simulink model "dt_universalUR16e_dh"  (R2026a)
settings: Solver=daessc  StopTime=2.50
undefined symbols (not defined in the file or in its folder): X, Y, Z
libraries: nesl_utility x29, sm_lib x25
settings Model: Creator=User  LastModifiedBy=User

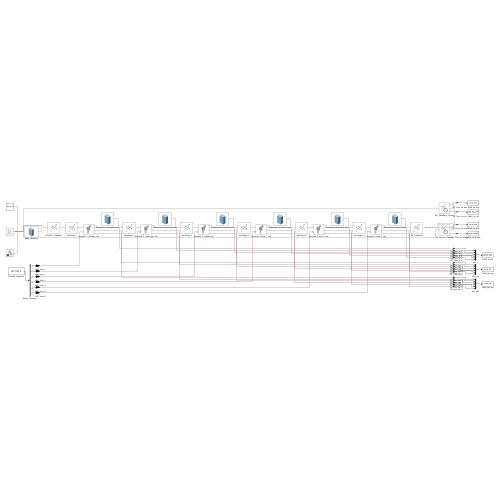
[thumbnail: Simulink's stored preview of the top-level diagram]
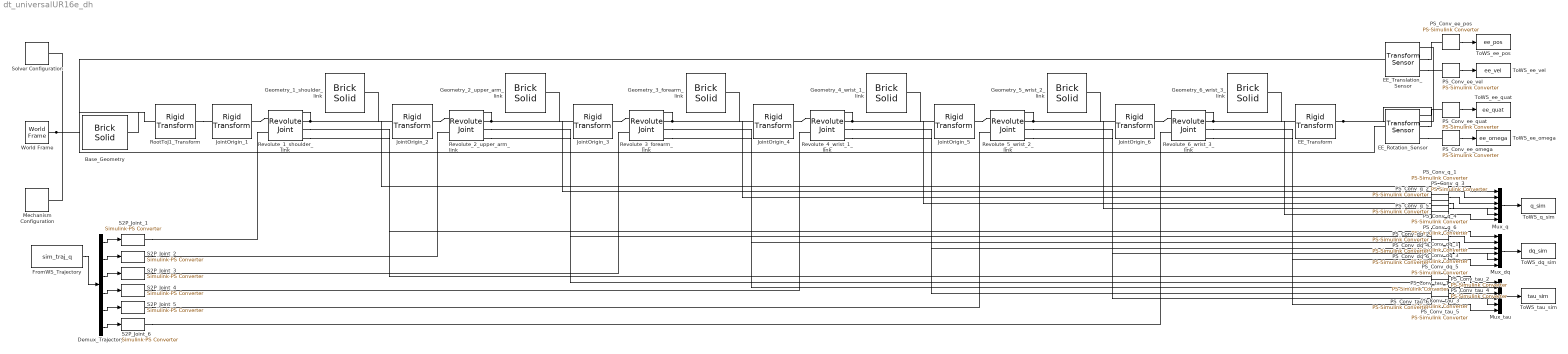
== system dt_universalUR16e_dh ==
  Base_Geometry : sm_lib/Body Elements/Brick Solid  BrickDimensions=[0.1, 0.1, 0.1]  BrickDimensionsUnits=m  ExportEntireGeometry=off  InertiaType=Custom  BasedOnType=Density  Density=1000  DensityUnits=kg/m^3  Mass=4.00000000  MassUnits=kg  CenterOfMass=[0.00000000, 0.00000000, 0.00000000]  CenterOfMassUnits=m  MomentsOfInertia=[0.00443000, 0.00443000, 0.00720000]  MomentsOfInertiaUnits=kg*m^2  ProductsOfInertia=[0, 0, 0]  ProductsOfInertiaUnits=kg*m^2  GraphicType=FromGeometry  MarkerShape=Sphere  MarkerSize=10  GraphicVisPropType=SimpleVisualProperties  GraphicDiffuseColor=[0.5 0.5 0.5]  GraphicOpacity=1  GraphicSpecularColor=[0.5 0.5 0.5 1.0]  GraphicAmbientColor=[0.15 0.15 0.15 1.0]  GraphicEmissiveColor=[0.0 0.0 0.0 1.0]  GraphicShininess=75  DoExposeReferenceFrame=on  SerializedFrames=<Frames/>
  Demux_Trajectory : Demux  Outputs=6
  EE_Rotation_Sensor : sm_lib/Frames and Transforms/Transform Sensor  MeasurementFrame=World  RotationSequence=XYX  SenseAngle=off  SenseAxis=off  SenseQ=on  SenseR=off  SenseRotationSequence=off  SenseOmegaX=off  SenseOmegaY=off  SenseOmegaZ=off  SenseOmega=on  SenseQDot=off  SenseRDot=off  SenseRotationSequenceDot=off  SenseAlphaX=off  SenseAlphaY=off  SenseAlphaZ=off  SenseAlpha=off  SenseQDDot=off  SenseRDDot=off  SenseX=off  SenseY=off  SenseZ=off  SenseXYZ=off  SenseRad=off  SenseAzim=off  SenseDist=off  SenseInc=off  SenseXDot=off  SenseYDot=off  SenseZDot=off  SenseXYZDot=off  SenseRadDot=off  SenseAzimDot=off  SenseDistDot=off  SenseIncDot=off  SenseXDDot=off  SenseYDDot=off  SenseZDDot=off  SenseXYZDDot=off  SenseRadDDot=off  SenseAzimDDot=off  SenseDistDDot=off  SenseIncDDot=off
  EE_Transform : sm_lib/Frames and Transforms/Rigid Transform  RotationMethod=ArbitraryAxis  FollAlignAxisA=+X  BaseAlignAxisA=+Y  FollAlignAxisB=+Y  BaseAlignAxisB=+Z  RotationStandardAxis=+Z  RotationAngle=3.1415926536  RotationAngleUnits=rad  RotationArbitraryAxis=[-0.0000000000, 1.0000000000, 0.0000000002]  RotationSequenceAxes=FollowerAxes  RotationSequence=XYX  RotationSequenceAngles=[0 0 0]  RotationSequenceAnglesUnits=deg  RotationMatrix=[1 0 0;0 1 0;0 0 1]  Quaternion=[1 0 0 0]  TranslationMethod=Cartesian  TranslationCartesianOffset=[-0.0000000000, -0.0000000000, -0.1165500000]  TranslationCartesianOffsetUnits=m  TranslationStandardAxis=+Z  TranslationStandardOffset=0  TranslationStandardOffsetUnits=m  TranslationROffset=0  TranslationROffsetUnits=m  TranslationThetaOffset=0  TranslationThetaOffsetUnits=deg  TranslationZOffset=0  TranslationZOffsetUnits=m
  EE_Translation_Sensor : sm_lib/Frames and Transforms/Transform Sensor  MeasurementFrame=World  RotationSequence=XYX  SenseAngle=off  SenseAxis=off  SenseQ=off  SenseR=off  SenseRotationSequence=off  SenseOmegaX=off  SenseOmegaY=off  SenseOmegaZ=off  SenseOmega=off  SenseQDot=off  SenseRDot=off  SenseRotationSequenceDot=off  SenseAlphaX=off  SenseAlphaY=off  SenseAlphaZ=off  SenseAlpha=off  SenseQDDot=off  SenseRDDot=off  SenseX=off  SenseY=off  SenseZ=off  SenseXYZ=on  SenseRad=off  SenseAzim=off  SenseDist=off  SenseInc=off  SenseXDot=off  SenseYDot=off  SenseZDot=off  SenseXYZDot=on  SenseRadDot=off  SenseAzimDot=off  SenseDistDot=off  SenseIncDot=off  SenseXDDot=off  SenseYDDot=off  SenseZDDot=off  SenseXYZDDot=off  SenseRadDDot=off  SenseAzimDDot=off  SenseDistDDot=off  SenseIncDDot=off
  FromWS_Trajectory : FromWorkspace  VariableName=sim_traj_q
  Geometry_1_shoulder_link : sm_lib/Body Elements/Brick Solid  BrickDimensions=[0.1, 0.1, 0.1]  BrickDimensionsUnits=m  ExportEntireGeometry=off  InertiaType=Custom  BasedOnType=Density  Density=1000  DensityUnits=kg/m^3  Mass=7.36900000  MassUnits=kg  CenterOfMass=[0.00000000, 0.00000000, 0.00000000]  CenterOfMassUnits=m  MomentsOfInertia=[0.02981926, 0.02981926, 0.02072531]  MomentsOfInertiaUnits=kg*m^2  ProductsOfInertia=[0.00000000, 0.00000000, 0.00000000]  ProductsOfInertiaUnits=kg*m^2  GraphicType=FromGeometry  MarkerShape=Sphere  MarkerSize=10  GraphicVisPropType=SimpleVisualProperties  GraphicDiffuseColor=[0.5 0.5 0.5]  GraphicOpacity=1  GraphicSpecularColor=[0.5 0.5 0.5 1.0]  GraphicAmbientColor=[0.15 0.15 0.15 1.0]  GraphicEmissiveColor=[0.0 0.0 0.0 1.0]  GraphicShininess=75  DoExposeReferenceFrame=on  SerializedFrames=<Frames/>
  Geometry_2_upper_arm_link : sm_lib/Body Elements/Brick Solid  BrickDimensions=[0.1, 0.1, 0.1]  BrickDimensionsUnits=m  ExportEntireGeometry=off  InertiaType=Custom  BasedOnType=Density  Density=1000  DensityUnits=kg/m^3  Mass=10.45000000  MassUnits=kg  CenterOfMass=[-0.23920000, 0.00000000, 0.17500000]  CenterOfMassUnits=m  MomentsOfInertia=[0.02939063, 0.21399986, 0.21399986]  MomentsOfInertiaUnits=kg*m^2  ProductsOfInertia=[0.00000000, -0.00000000, 0.00000000]  ProductsOfInertiaUnits=kg*m^2  GraphicType=FromGeometry  MarkerShape=Sphere  MarkerSize=10  GraphicVisPropType=SimpleVisualProperties  GraphicDiffuseColor=[0.5 0.5 0.5]  GraphicOpacity=1  GraphicSpecularColor=[0.5 0.5 0.5 1.0]  GraphicAmbientColor=[0.15 0.15 0.15 1.0]  GraphicEmissiveColor=[0.0 0.0 0.0 1.0]  GraphicShininess=75  DoExposeReferenceFrame=on  SerializedFrames=<Frames/>
  Geometry_3_forearm_link : sm_lib/Body Elements/Brick Solid  BrickDimensions=[0.1, 0.1, 0.1]  BrickDimensionsUnits=m  ExportEntireGeometry=off  InertiaType=Custom  BasedOnType=Density  Density=1000  DensityUnits=kg/m^3  Mass=4.32100000  MassUnits=kg  CenterOfMass=[-0.18000000, 0.00000000, 0.04000000]  CenterOfMassUnits=m  MomentsOfInertia=[0.01215281, 0.05274319, 0.05274319]  MomentsOfInertiaUnits=kg*m^2  ProductsOfInertia=[0.00000000, -0.00000000, 0.00000000]  ProductsOfInertiaUnits=kg*m^2  GraphicType=FromGeometry  MarkerShape=Sphere  MarkerSize=10  GraphicVisPropType=SimpleVisualProperties  GraphicDiffuseColor=[0.5 0.5 0.5]  GraphicOpacity=1  GraphicSpecularColor=[0.5 0.5 0.5 1.0]  GraphicAmbientColor=[0.15 0.15 0.15 1.0]  GraphicEmissiveColor=[0.0 0.0 0.0 1.0]  GraphicShininess=75  DoExposeReferenceFrame=on  SerializedFrames=<Frames/>
  Geometry_4_wrist_1_link : sm_lib/Body Elements/Brick Solid  BrickDimensions=[0.1, 0.1, 0.1]  BrickDimensionsUnits=m  ExportEntireGeometry=off  InertiaType=Custom  BasedOnType=Density  Density=1000  DensityUnits=kg/m^3  Mass=2.18000000  MassUnits=kg  CenterOfMass=[0.00000000, 0.00000000, 0.00000000]  CenterOfMassUnits=m  MomentsOfInertia=[0.00568162, 0.00568162, 0.00613125]  MomentsOfInertiaUnits=kg*m^2  ProductsOfInertia=[0.00000000, 0.00000000, 0.00000000]  ProductsOfInertiaUnits=kg*m^2  GraphicType=FromGeometry  MarkerShape=Sphere  MarkerSize=10  GraphicVisPropType=SimpleVisualProperties  GraphicDiffuseColor=[0.5 0.5 0.5]  GraphicOpacity=1  GraphicSpecularColor=[0.5 0.5 0.5 1.0]  GraphicAmbientColor=[0.15 0.15 0.15 1.0]  GraphicEmissiveColor=[0.0 0.0 0.0 1.0]  GraphicShininess=75  DoExposeReferenceFrame=on  SerializedFrames=<Frames/>
  Geometry_5_wrist_2_link : sm_lib/Body Elements/Brick Solid  BrickDimensions=[0.1, 0.1, 0.1]  BrickDimensionsUnits=m  ExportEntireGeometry=off  InertiaType=Custom  BasedOnType=Density  Density=1000  DensityUnits=kg/m^3  Mass=2.03300000  MassUnits=kg  CenterOfMass=[0.00000000, 0.00000000, 0.00000000]  CenterOfMassUnits=m  MomentsOfInertia=[0.00529850, 0.00529850, 0.00571781]  MomentsOfInertiaUnits=kg*m^2  ProductsOfInertia=[0.00000000, 0.00000000, 0.00000000]  ProductsOfInertiaUnits=kg*m^2  GraphicType=FromGeometry  MarkerShape=Sphere  MarkerSize=10  GraphicVisPropType=SimpleVisualProperties  GraphicDiffuseColor=[0.5 0.5 0.5]  GraphicOpacity=1  GraphicSpecularColor=[0.5 0.5 0.5 1.0]  GraphicAmbientColor=[0.15 0.15 0.15 1.0]  GraphicEmissiveColor=[0.0 0.0 0.0 1.0]  GraphicShininess=75  DoExposeReferenceFrame=on  SerializedFrames=<Frames/>
  Geometry_6_wrist_3_link : sm_lib/Body Elements/Brick Solid  BrickDimensions=[0.1, 0.1, 0.1]  BrickDimensionsUnits=m  ExportEntireGeometry=off  InertiaType=Custom  BasedOnType=Density  Density=1000  DensityUnits=kg/m^3  Mass=0.90700000  MassUnits=kg  CenterOfMass=[0.00000000, 0.00000000, -0.02500000]  CenterOfMassUnits=m  MomentsOfInertia=[0.00064813, 0.00064813, 0.00091834]  MomentsOfInertiaUnits=kg*m^2  ProductsOfInertia=[0.00000000, 0.00000000, 0.00000000]  ProductsOfInertiaUnits=kg*m^2  GraphicType=FromGeometry  MarkerShape=Sphere  MarkerSize=10  GraphicVisPropType=SimpleVisualProperties  GraphicDiffuseColor=[0.5 0.5 0.5]  GraphicOpacity=1  GraphicSpecularColor=[0.5 0.5 0.5 1.0]  GraphicAmbientColor=[0.15 0.15 0.15 1.0]  GraphicEmissiveColor=[0.0 0.0 0.0 1.0]  GraphicShininess=75  DoExposeReferenceFrame=on  SerializedFrames=<Frames/>
  JointOrigin_1 : sm_lib/Frames and Transforms/Rigid Transform  RotationMethod=None  FollAlignAxisA=+X  BaseAlignAxisA=+Y  FollAlignAxisB=+Y  BaseAlignAxisB=+Z  RotationStandardAxis=+Z  RotationAngle=0  RotationAngleUnits=deg  RotationArbitraryAxis=[0 0 1]  RotationSequenceAxes=FollowerAxes  RotationSequence=XYX  RotationSequenceAngles=[0 0 0]  RotationSequenceAnglesUnits=deg  RotationMatrix=[1 0 0;0 1 0;0 0 1]  Quaternion=[1 0 0 0]  TranslationMethod=Cartesian  TranslationCartesianOffset=[0.0000000000, 0.0000000000, 0.1807000000]  TranslationCartesianOffsetUnits=m  TranslationStandardAxis=+Z  TranslationStandardOffset=0  TranslationStandardOffsetUnits=m  TranslationROffset=0  TranslationROffsetUnits=m  TranslationThetaOffset=0  TranslationThetaOffsetUnits=deg  TranslationZOffset=0  TranslationZOffsetUnits=m
  JointOrigin_2 : sm_lib/Frames and Transforms/Rigid Transform  RotationMethod=ArbitraryAxis  FollAlignAxisA=+X  BaseAlignAxisA=+Y  FollAlignAxisB=+Y  BaseAlignAxisB=+Z  RotationStandardAxis=+Z  RotationAngle=1.5707963270  RotationAngleUnits=rad  RotationArbitraryAxis=[1.0000000000, 0.0000000000, 0.0000000000]  RotationSequenceAxes=FollowerAxes  RotationSequence=XYX  RotationSequenceAngles=[0 0 0]  RotationSequenceAnglesUnits=deg  RotationMatrix=[1 0 0;0 1 0;0 0 1]  Quaternion=[1 0 0 0]  TranslationMethod=Cartesian  TranslationCartesianOffset=[0.0000000000, 0.0000000000, 0.0000000000]  TranslationCartesianOffsetUnits=m  TranslationStandardAxis=+Z  TranslationStandardOffset=0  TranslationStandardOffsetUnits=m  TranslationROffset=0  TranslationROffsetUnits=m  TranslationThetaOffset=0  TranslationThetaOffsetUnits=deg  TranslationZOffset=0  TranslationZOffsetUnits=m
  JointOrigin_3 : sm_lib/Frames and Transforms/Rigid Transform  RotationMethod=None  FollAlignAxisA=+X  BaseAlignAxisA=+Y  FollAlignAxisB=+Y  BaseAlignAxisB=+Z  RotationStandardAxis=+Z  RotationAngle=0  RotationAngleUnits=deg  RotationArbitraryAxis=[0 0 1]  RotationSequenceAxes=FollowerAxes  RotationSequence=XYX  RotationSequenceAngles=[0 0 0]  RotationSequenceAnglesUnits=deg  RotationMatrix=[1 0 0;0 1 0;0 0 1]  Quaternion=[1 0 0 0]  TranslationMethod=Cartesian  TranslationCartesianOffset=[-0.4784000000, 0.0000000000, 0.0000000000]  TranslationCartesianOffsetUnits=m  TranslationStandardAxis=+Z  TranslationStandardOffset=0  TranslationStandardOffsetUnits=m  TranslationROffset=0  TranslationROffsetUnits=m  TranslationThetaOffset=0  TranslationThetaOffsetUnits=deg  TranslationZOffset=0  TranslationZOffsetUnits=m
  JointOrigin_4 : sm_lib/Frames and Transforms/Rigid Transform  RotationMethod=None  FollAlignAxisA=+X  BaseAlignAxisA=+Y  FollAlignAxisB=+Y  BaseAlignAxisB=+Z  RotationStandardAxis=+Z  RotationAngle=0  RotationAngleUnits=deg  RotationArbitraryAxis=[0 0 1]  RotationSequenceAxes=FollowerAxes  RotationSequence=XYX  RotationSequenceAngles=[0 0 0]  RotationSequenceAnglesUnits=deg  RotationMatrix=[1 0 0;0 1 0;0 0 1]  Quaternion=[1 0 0 0]  TranslationMethod=Cartesian  TranslationCartesianOffset=[-0.3600000000, 0.0000000000, 0.1741500000]  TranslationCartesianOffsetUnits=m  TranslationStandardAxis=+Z  TranslationStandardOffset=0  TranslationStandardOffsetUnits=m  TranslationROffset=0  TranslationROffsetUnits=m  TranslationThetaOffset=0  TranslationThetaOffsetUnits=deg  TranslationZOffset=0  TranslationZOffsetUnits=m
  JointOrigin_5 : sm_lib/Frames and Transforms/Rigid Transform  RotationMethod=ArbitraryAxis  FollAlignAxisA=+X  BaseAlignAxisA=+Y  FollAlignAxisB=+Y  BaseAlignAxisB=+Z  RotationStandardAxis=+Z  RotationAngle=1.5707963270  RotationAngleUnits=rad  RotationArbitraryAxis=[1.0000000000, 0.0000000000, 0.0000000000]  RotationSequenceAxes=FollowerAxes  RotationSequence=XYX  RotationSequenceAngles=[0 0 0]  RotationSequenceAnglesUnits=deg  RotationMatrix=[1 0 0;0 1 0;0 0 1]  Quaternion=[1 0 0 0]  TranslationMethod=Cartesian  TranslationCartesianOffset=[0.0000000000, -0.1198500000, -0.0000000000]  TranslationCartesianOffsetUnits=m  TranslationStandardAxis=+Z  TranslationStandardOffset=0  TranslationStandardOffsetUnits=m  TranslationROffset=0  TranslationROffsetUnits=m  TranslationThetaOffset=0  TranslationThetaOffsetUnits=deg  TranslationZOffset=0  TranslationZOffsetUnits=m
  JointOrigin_6 : sm_lib/Frames and Transforms/Rigid Transform  RotationMethod=ArbitraryAxis  FollAlignAxisA=+X  BaseAlignAxisA=+Y  FollAlignAxisB=+Y  BaseAlignAxisB=+Z  RotationStandardAxis=+Z  RotationAngle=1.5707963270  RotationAngleUnits=rad  RotationArbitraryAxis=[-1.0000000000, -0.0000000000, -0.0000000000]  RotationSequenceAxes=FollowerAxes  RotationSequence=XYX  RotationSequenceAngles=[0 0 0]  RotationSequenceAnglesUnits=deg  RotationMatrix=[1 0 0;0 1 0;0 0 1]  Quaternion=[1 0 0 0]  TranslationMethod=Cartesian  TranslationCartesianOffset=[0.0000000000, 0.1165500000, -0.0000000000]  TranslationCartesianOffsetUnits=m  TranslationStandardAxis=+Z  TranslationStandardOffset=0  TranslationStandardOffsetUnits=m  TranslationROffset=0  TranslationROffsetUnits=m  TranslationThetaOffset=0  TranslationThetaOffsetUnits=deg  TranslationZOffset=0  TranslationZOffsetUnits=m
  Mechanism Configuration : sm_lib/Utilities/Mechanism Configuration  UniformGravity=Constant  GravityVector=[0.0000000000, 0.0000000000, -9.8100000000]  GravityVectorUnits=m/s^2  LinearizationDelta=0.001  JointModeTransitionNonlinearIterations=2
  Mux_dq : Mux  Inputs=6
  Mux_q : Mux  Inputs=6
  Mux_tau : Mux  Inputs=6
  PS_Conv_dq_{1..6} (6 alike) : nesl_utility/PS-Simulink Converter  PhysicalDomain=network_engine_domain  SubClassName=ps_output  LeftPortType=input  RightPortType=output  PseudoPeriodic=off  Frequencies=[]  VectorFormat=inherit  Unit=inherit  AffineConversion=off
  PS_Conv_ee_omega : nesl_utility/PS-Simulink Converter  PhysicalDomain=network_engine_domain  SubClassName=ps_output  LeftPortType=input  RightPortType=output  PseudoPeriodic=off  Frequencies=[]  VectorFormat=inherit  Unit=inherit  AffineConversion=off
  PS_Conv_ee_pos : nesl_utility/PS-Simulink Converter  PhysicalDomain=network_engine_domain  SubClassName=ps_output  LeftPortType=input  RightPortType=output  PseudoPeriodic=off  Frequencies=[]  VectorFormat=inherit  Unit=inherit  AffineConversion=off
  PS_Conv_ee_quat : nesl_utility/PS-Simulink Converter  PhysicalDomain=network_engine_domain  SubClassName=ps_output  LeftPortType=input  RightPortType=output  PseudoPeriodic=off  Frequencies=[]  VectorFormat=inherit  Unit=inherit  AffineConversion=off
  PS_Conv_ee_vel : nesl_utility/PS-Simulink Converter  PhysicalDomain=network_engine_domain  SubClassName=ps_output  LeftPortType=input  RightPortType=output  PseudoPeriodic=off  Frequencies=[]  VectorFormat=inherit  Unit=inherit  AffineConversion=off
  PS_Conv_q_{1..6} (6 alike) : nesl_utility/PS-Simulink Converter  PhysicalDomain=network_engine_domain  SubClassName=ps_output  LeftPortType=input  RightPortType=output  PseudoPeriodic=off  Frequencies=[]  VectorFormat=inherit  Unit=inherit  AffineConversion=off
  PS_Conv_tau_{1..6} (6 alike) : nesl_utility/PS-Simulink Converter  PhysicalDomain=network_engine_domain  SubClassName=ps_output  LeftPortType=input  RightPortType=output  PseudoPeriodic=off  Frequencies=[]  VectorFormat=inherit  Unit=inherit  AffineConversion=off
  Revolute_1_shoulder_link : sm_lib/Joints/Revolute Joint  JointMode=Normal  CompositeWrenchDir=FollowerOnBase  CompositeWrenchFrame=BaseFrame  SenseConstraintForce=off  SenseConstraintTorque=off  SenseTotalForce=off  SenseTotalTorque=off  PositionTargetSpecify=off  PositionTargetPriority=High  PositionTargetValue=0  PositionTargetValueUnits=deg  VelocityTargetSpecify=off  VelocityTargetPriority=High  VelocityTargetValue=0  VelocityTargetValueUnits=deg/s  EquilibriumPosition=0  EquilibriumPositionUnits=deg  SpringStiffness=0  SpringStiffnessUnits=N*m/deg  DampingCoefficient=0  DampingCoefficientUnits=N*m/(deg/s)  LowerLimitSpecify=off  LowerLimitBound=-90  LowerLimitBoundUnits=deg  LowerLimitStiffness=1e4  LowerLimitStiffnessUnits=N*m/deg  LowerLimitDamping=10  LowerLimitDampingUnits=N*m/(deg/s)  LowerLimitTransitionRegionWidth=0.1  LowerLimitTransitionRegionWidthUnits=deg  UpperLimitSpecify=off  UpperLimitBound=90  UpperLimitBoundUnits=deg  UpperLimitStiffness=1e4  UpperLimitStiffnessUnits=N*m/deg  UpperLimitDamping=10  UpperLimitDampingUnits=N*m/(deg/s)  UpperLimitTransitionRegionWidth=0.1  UpperLimitTransitionRegionWidthUnits=deg  TorqueActuationMode=ComputedTorque  MotionActuationMode=InputMotion  SensePosition=on  SenseVelocity=on  SenseAcceleration=off  SenseTorqueForce=on  SenseLowerLimitTorqueForce=off  SenseUpperLimitTorqueForce=off
  Revolute_2_upper_arm_link : sm_lib/Joints/Revolute Joint  JointMode=Normal  CompositeWrenchDir=FollowerOnBase  CompositeWrenchFrame=BaseFrame  SenseConstraintForce=off  SenseConstraintTorque=off  SenseTotalForce=off  SenseTotalTorque=off  PositionTargetSpecify=off  PositionTargetPriority=High  PositionTargetValue=0  PositionTargetValueUnits=deg  VelocityTargetSpecify=off  VelocityTargetPriority=High  VelocityTargetValue=0  VelocityTargetValueUnits=deg/s  EquilibriumPosition=0  EquilibriumPositionUnits=deg  SpringStiffness=0  SpringStiffnessUnits=N*m/deg  DampingCoefficient=0  DampingCoefficientUnits=N*m/(deg/s)  LowerLimitSpecify=off  LowerLimitBound=-90  LowerLimitBoundUnits=deg  LowerLimitStiffness=1e4  LowerLimitStiffnessUnits=N*m/deg  LowerLimitDamping=10  LowerLimitDampingUnits=N*m/(deg/s)  LowerLimitTransitionRegionWidth=0.1  LowerLimitTransitionRegionWidthUnits=deg  UpperLimitSpecify=off  UpperLimitBound=90  UpperLimitBoundUnits=deg  UpperLimitStiffness=1e4  UpperLimitStiffnessUnits=N*m/deg  UpperLimitDamping=10  UpperLimitDampingUnits=N*m/(deg/s)  UpperLimitTransitionRegionWidth=0.1  UpperLimitTransitionRegionWidthUnits=deg  TorqueActuationMode=ComputedTorque  MotionActuationMode=InputMotion  SensePosition=on  SenseVelocity=on  SenseAcceleration=off  SenseTorqueForce=on  SenseLowerLimitTorqueForce=off  SenseUpperLimitTorqueForce=off
  Revolute_3_forearm_link : sm_lib/Joints/Revolute Joint  JointMode=Normal  CompositeWrenchDir=FollowerOnBase  CompositeWrenchFrame=BaseFrame  SenseConstraintForce=off  SenseConstraintTorque=off  SenseTotalForce=off  SenseTotalTorque=off  PositionTargetSpecify=off  PositionTargetPriority=High  PositionTargetValue=0  PositionTargetValueUnits=deg  VelocityTargetSpecify=off  VelocityTargetPriority=High  VelocityTargetValue=0  VelocityTargetValueUnits=deg/s  EquilibriumPosition=0  EquilibriumPositionUnits=deg  SpringStiffness=0  SpringStiffnessUnits=N*m/deg  DampingCoefficient=0  DampingCoefficientUnits=N*m/(deg/s)  LowerLimitSpecify=off  LowerLimitBound=-90  LowerLimitBoundUnits=deg  LowerLimitStiffness=1e4  LowerLimitStiffnessUnits=N*m/deg  LowerLimitDamping=10  LowerLimitDampingUnits=N*m/(deg/s)  LowerLimitTransitionRegionWidth=0.1  LowerLimitTransitionRegionWidthUnits=deg  UpperLimitSpecify=off  UpperLimitBound=90  UpperLimitBoundUnits=deg  UpperLimitStiffness=1e4  UpperLimitStiffnessUnits=N*m/deg  UpperLimitDamping=10  UpperLimitDampingUnits=N*m/(deg/s)  UpperLimitTransitionRegionWidth=0.1  UpperLimitTransitionRegionWidthUnits=deg  TorqueActuationMode=ComputedTorque  MotionActuationMode=InputMotion  SensePosition=on  SenseVelocity=on  SenseAcceleration=off  SenseTorqueForce=on  SenseLowerLimitTorqueForce=off  SenseUpperLimitTorqueForce=off
  Revolute_4_wrist_1_link : sm_lib/Joints/Revolute Joint  JointMode=Normal  CompositeWrenchDir=FollowerOnBase  CompositeWrenchFrame=BaseFrame  SenseConstraintForce=off  SenseConstraintTorque=off  SenseTotalForce=off  SenseTotalTorque=off  PositionTargetSpecify=off  PositionTargetPriority=High  PositionTargetValue=0  PositionTargetValueUnits=deg  VelocityTargetSpecify=off  VelocityTargetPriority=High  VelocityTargetValue=0  VelocityTargetValueUnits=deg/s  EquilibriumPosition=0  EquilibriumPositionUnits=deg  SpringStiffness=0  SpringStiffnessUnits=N*m/deg  DampingCoefficient=0  DampingCoefficientUnits=N*m/(deg/s)  LowerLimitSpecify=off  LowerLimitBound=-90  LowerLimitBoundUnits=deg  LowerLimitStiffness=1e4  LowerLimitStiffnessUnits=N*m/deg  LowerLimitDamping=10  LowerLimitDampingUnits=N*m/(deg/s)  LowerLimitTransitionRegionWidth=0.1  LowerLimitTransitionRegionWidthUnits=deg  UpperLimitSpecify=off  UpperLimitBound=90  UpperLimitBoundUnits=deg  UpperLimitStiffness=1e4  UpperLimitStiffnessUnits=N*m/deg  UpperLimitDamping=10  UpperLimitDampingUnits=N*m/(deg/s)  UpperLimitTransitionRegionWidth=0.1  UpperLimitTransitionRegionWidthUnits=deg  TorqueActuationMode=ComputedTorque  MotionActuationMode=InputMotion  SensePosition=on  SenseVelocity=on  SenseAcceleration=off  SenseTorqueForce=on  SenseLowerLimitTorqueForce=off  SenseUpperLimitTorqueForce=off
  Revolute_5_wrist_2_link : sm_lib/Joints/Revolute Joint  JointMode=Normal  CompositeWrenchDir=FollowerOnBase  CompositeWrenchFrame=BaseFrame  SenseConstraintForce=off  SenseConstraintTorque=off  SenseTotalForce=off  SenseTotalTorque=off  PositionTargetSpecify=off  PositionTargetPriority=High  PositionTargetValue=0  PositionTargetValueUnits=deg  VelocityTargetSpecify=off  VelocityTargetPriority=High  VelocityTargetValue=0  VelocityTargetValueUnits=deg/s  EquilibriumPosition=0  EquilibriumPositionUnits=deg  SpringStiffness=0  SpringStiffnessUnits=N*m/deg  DampingCoefficient=0  DampingCoefficientUnits=N*m/(deg/s)  LowerLimitSpecify=off  LowerLimitBound=-90  LowerLimitBoundUnits=deg  LowerLimitStiffness=1e4  LowerLimitStiffnessUnits=N*m/deg  LowerLimitDamping=10  LowerLimitDampingUnits=N*m/(deg/s)  LowerLimitTransitionRegionWidth=0.1  LowerLimitTransitionRegionWidthUnits=deg  UpperLimitSpecify=off  UpperLimitBound=90  UpperLimitBoundUnits=deg  UpperLimitStiffness=1e4  UpperLimitStiffnessUnits=N*m/deg  UpperLimitDamping=10  UpperLimitDampingUnits=N*m/(deg/s)  UpperLimitTransitionRegionWidth=0.1  UpperLimitTransitionRegionWidthUnits=deg  TorqueActuationMode=ComputedTorque  MotionActuationMode=InputMotion  SensePosition=on  SenseVelocity=on  SenseAcceleration=off  SenseTorqueForce=on  SenseLowerLimitTorqueForce=off  SenseUpperLimitTorqueForce=off
  Revolute_6_wrist_3_link : sm_lib/Joints/Revolute Joint  JointMode=Normal  CompositeWrenchDir=FollowerOnBase  CompositeWrenchFrame=BaseFrame  SenseConstraintForce=off  SenseConstraintTorque=off  SenseTotalForce=off  SenseTotalTorque=off  PositionTargetSpecify=off  PositionTargetPriority=High  PositionTargetValue=0  PositionTargetValueUnits=deg  VelocityTargetSpecify=off  VelocityTargetPriority=High  VelocityTargetValue=0  VelocityTargetValueUnits=deg/s  EquilibriumPosition=0  EquilibriumPositionUnits=deg  SpringStiffness=0  SpringStiffnessUnits=N*m/deg  DampingCoefficient=0  DampingCoefficientUnits=N*m/(deg/s)  LowerLimitSpecify=off  LowerLimitBound=-90  LowerLimitBoundUnits=deg  LowerLimitStiffness=1e4  LowerLimitStiffnessUnits=N*m/deg  LowerLimitDamping=10  LowerLimitDampingUnits=N*m/(deg/s)  LowerLimitTransitionRegionWidth=0.1  LowerLimitTransitionRegionWidthUnits=deg  UpperLimitSpecify=off  UpperLimitBound=90  UpperLimitBoundUnits=deg  UpperLimitStiffness=1e4  UpperLimitStiffnessUnits=N*m/deg  UpperLimitDamping=10  UpperLimitDampingUnits=N*m/(deg/s)  UpperLimitTransitionRegionWidth=0.1  UpperLimitTransitionRegionWidthUnits=deg  TorqueActuationMode=ComputedTorque  MotionActuationMode=InputMotion  SensePosition=on  SenseVelocity=on  SenseAcceleration=off  SenseTorqueForce=on  SenseLowerLimitTorqueForce=off  SenseUpperLimitTorqueForce=off
  RootToJ1_Transform : sm_lib/Frames and Transforms/Rigid Transform  RotationMethod=ArbitraryAxis  FollAlignAxisA=+X  BaseAlignAxisA=+Y  FollAlignAxisB=+Y  BaseAlignAxisB=+Z  RotationStandardAxis=+Z  RotationAngle=3.1415926536  RotationAngleUnits=rad  RotationArbitraryAxis=[0.0000000000, 0.0000000000, 1.0000000000]  RotationSequenceAxes=FollowerAxes  RotationSequence=XYX  RotationSequenceAngles=[0 0 0]  RotationSequenceAnglesUnits=deg  RotationMatrix=[1 0 0;0 1 0;0 0 1]  Quaternion=[1 0 0 0]  TranslationMethod=Cartesian  TranslationCartesianOffset=[0.0000000000, 0.0000000000, 0.0000000000]  TranslationCartesianOffsetUnits=m  TranslationStandardAxis=+Z  TranslationStandardOffset=0  TranslationStandardOffsetUnits=m  TranslationROffset=0  TranslationROffsetUnits=m  TranslationThetaOffset=0  TranslationThetaOffsetUnits=deg  TranslationZOffset=0  TranslationZOffsetUnits=m
  S2P_Joint_{1..6} (6 alike) : nesl_utility/Simulink-PS Converter  PhysicalDomain=network_engine_domain  SubClassName=ps_input  LeftPortType=input  RightPortType=output  PseudoPeriodic=off  Frequencies=[]  NoiseDistribution=none  NoiseParameters=[]  Unit=rad  AffineConversion=off  FilteringAndDerivatives=filter  SimscapeFilterOrder=2  InputFilterTimeConstant=0.0002  UdotUserProvided=0
  Solver Configuration : nesl_utility/Solver Configuration  PhysicalDomain=network_engine_domain  SubClassName=solver  LeftPortType=input  RightPortType=generic  Tones=[]  Harmonics=[]  SimulateNoise=off  Profile=off  UseLocalSampling=off  EnableSwitchedLinearOptims=on  FrequencyDomain=off  UseCCode=off  RelTol=0.001  AbsTol=0.001  MinStep=1e-09  ToWorkspace=off  RevertToSquareIcSolve=off  NumHomotopyIterations=100  PhasorMode=off  PhasorModeNumHarmonics=1  ConsistencySolver=NEWTON_XTOL_AFTER_FTOL  CanonicalOrdering=CANONICAL  OptimizeIntermediates=OPTIMIZED  IndexReductionMethod=DerivativeReplacement  DoDC=off  ResidualTolerance=1e-09  ConsistencyTolSource=GLOBAL  ConsistencyAbsTol=0.001  ConsistencyRelTol=0.001  ConsistencyTolFactor=0.001  UseLocalSolver=off  LocalSolverChoice=NE_BACKWARD_EULER_ADVANCER  ResolveIndetEquations=on  FunctionEvalNumThread=1  LocalSolverSampleTime=0.001  DoFixedCost=off  MaxNonlinIter=3  MaxModeIter=2  ComputeImpulses=off  ImpulseIterations=2  LinearAlgebra=auto  LinearAlgebraNumThread=0  EquationFormulation=NE_TIME_EF  DelaysMemoryBudget=1024  AutomaticFiltering=on  FilteringTimeConstant=0.001  PartitionStorageMethod=AS_NEEDED  PartitionMemoryBudget=1024  PartitionMethod=ROBUST  MultibodyUseLocalSolver=off  MultibodyLocalSolverChoice=ODE1  MultibodyLocalSolverSampleTime=0.001
  ToWS_dq_sim : ToWorkspace  VariableName=dq_sim  SaveFormat=Timeseries  SampleTime=-1
  ToWS_ee_omega : ToWorkspace  VariableName=ee_omega  SaveFormat=Timeseries  SampleTime=-1
  ToWS_ee_pos : ToWorkspace  VariableName=ee_pos  SaveFormat=Timeseries  SampleTime=-1
  ToWS_ee_quat : ToWorkspace  VariableName=ee_quat  SaveFormat=Timeseries  SampleTime=-1
  ToWS_ee_vel : ToWorkspace  VariableName=ee_vel  SaveFormat=Timeseries  SampleTime=-1
  ToWS_q_sim : ToWorkspace  VariableName=q_sim  SaveFormat=Timeseries  SampleTime=-1
  ToWS_tau_sim : ToWorkspace  VariableName=tau_sim  SaveFormat=Timeseries  SampleTime=-1
  World Frame : sm_lib/Frames and Transforms/World Frame
  wires:
  PS_Conv_ee_pos/1 -> ToWS_ee_pos/1
  PS_Conv_ee_vel/1 -> ToWS_ee_vel/1
  PS_Conv_ee_quat/1 -> ToWS_ee_quat/1
  PS_Conv_ee_omega/1 -> ToWS_ee_omega/1
  PS_Conv_q_1/1 -> Mux_q/1
  PS_Conv_dq_1/1 -> Mux_dq/1
  PS_Conv_tau_1/1 -> Mux_tau/1
  PS_Conv_q_2/1 -> Mux_q/2
  PS_Conv_dq_2/1 -> Mux_dq/2
  PS_Conv_tau_2/1 -> Mux_tau/2
  PS_Conv_q_3/1 -> Mux_q/3
  PS_Conv_dq_3/1 -> Mux_dq/3
  PS_Conv_tau_3/1 -> Mux_tau/3
  PS_Conv_q_4/1 -> Mux_q/4
  PS_Conv_dq_4/1 -> Mux_dq/4
  PS_Conv_tau_4/1 -> Mux_tau/4
  PS_Conv_q_5/1 -> Mux_q/5
  PS_Conv_dq_5/1 -> Mux_dq/5
  PS_Conv_tau_5/1 -> Mux_tau/5
  PS_Conv_q_6/1 -> Mux_q/6
  PS_Conv_dq_6/1 -> Mux_dq/6
  PS_Conv_tau_6/1 -> Mux_tau/6
  Mux_q/1 -> ToWS_q_sim/1
  Mux_dq/1 -> ToWS_dq_sim/1
  Mux_tau/1 -> ToWS_tau_sim/1
  FromWS_Trajectory/1 -> Demux_Trajectory/1
  Demux_Trajectory/1 -> S2P_Joint_1/1
  Demux_Trajectory/2 -> S2P_Joint_2/1
  Demux_Trajectory/3 -> S2P_Joint_3/1
  Demux_Trajectory/4 -> S2P_Joint_4/1
  Demux_Trajectory/5 -> S2P_Joint_5/1
  Demux_Trajectory/6 -> S2P_Joint_6/1
  connections:
  Solver Configuration/RConn1 -- World Frame/RConn1 -- Mechanism Configuration/RConn1 -- Base_Geometry/RConn1 -- RootToJ1_Transform/LConn1 -- EE_Translation_Sensor/LConn1 -- EE_Rotation_Sensor/LConn1
  RootToJ1_Transform/RConn1 -- JointOrigin_1/LConn1
  JointOrigin_1/RConn1 -- Revolute_1_shoulder_link/LConn1
  Geometry_1_shoulder_link/RConn1 -- Revolute_1_shoulder_link/RConn1 -- JointOrigin_2/LConn1
  JointOrigin_2/RConn1 -- Revolute_2_upper_arm_link/LConn1
  Geometry_2_upper_arm_link/RConn1 -- Revolute_2_upper_arm_link/RConn1 -- JointOrigin_3/LConn1
  JointOrigin_3/RConn1 -- Revolute_3_forearm_link/LConn1
  Geometry_3_forearm_link/RConn1 -- Revolute_3_forearm_link/RConn1 -- JointOrigin_4/LConn1
  JointOrigin_4/RConn1 -- Revolute_4_wrist_1_link/LConn1
  Geometry_4_wrist_1_link/RConn1 -- Revolute_4_wrist_1_link/RConn1 -- JointOrigin_5/LConn1
  JointOrigin_5/RConn1 -- Revolute_5_wrist_2_link/LConn1
  Geometry_5_wrist_2_link/RConn1 -- Revolute_5_wrist_2_link/RConn1 -- JointOrigin_6/LConn1
  JointOrigin_6/RConn1 -- Revolute_6_wrist_3_link/LConn1
  Geometry_6_wrist_3_link/RConn1 -- Revolute_6_wrist_3_link/RConn1 -- EE_Transform/LConn1
  EE_Translation_Sensor/RConn1 -- EE_Transform/RConn1 -- EE_Rotation_Sensor/RConn1
  EE_Translation_Sensor/RConn2 -- PS_Conv_ee_pos/LConn1
  EE_Translation_Sensor/RConn3 -- PS_Conv_ee_vel/LConn1
  EE_Rotation_Sensor/RConn2 -- PS_Conv_ee_quat/LConn1
  EE_Rotation_Sensor/RConn3 -- PS_Conv_ee_omega/LConn1
  Revolute_1_shoulder_link/RConn2 -- PS_Conv_q_1/LConn1
  Revolute_1_shoulder_link/RConn3 -- PS_Conv_dq_1/LConn1
  Revolute_1_shoulder_link/RConn4 -- PS_Conv_tau_1/LConn1
  Revolute_2_upper_arm_link/RConn2 -- PS_Conv_q_2/LConn1
  Revolute_2_upper_arm_link/RConn3 -- PS_Conv_dq_2/LConn1
  Revolute_2_upper_arm_link/RConn4 -- PS_Conv_tau_2/LConn1
  Revolute_3_forearm_link/RConn2 -- PS_Conv_q_3/LConn1
  Revolute_3_forearm_link/RConn3 -- PS_Conv_dq_3/LConn1
  Revolute_3_forearm_link/RConn4 -- PS_Conv_tau_3/LConn1
  Revolute_4_wrist_1_link/RConn2 -- PS_Conv_q_4/LConn1
  Revolute_4_wrist_1_link/RConn3 -- PS_Conv_dq_4/LConn1
  Revolute_4_wrist_1_link/RConn4 -- PS_Conv_tau_4/LConn1
  Revolute_5_wrist_2_link/RConn2 -- PS_Conv_q_5/LConn1
  Revolute_5_wrist_2_link/RConn3 -- PS_Conv_dq_5/LConn1
  Revolute_5_wrist_2_link/RConn4 -- PS_Conv_tau_5/LConn1
  Revolute_6_wrist_3_link/RConn2 -- PS_Conv_q_6/LConn1
  Revolute_6_wrist_3_link/RConn3 -- PS_Conv_dq_6/LConn1
  Revolute_6_wrist_3_link/RConn4 -- PS_Conv_tau_6/LConn1
  S2P_Joint_1/RConn1 -- Revolute_1_shoulder_link/LConn2
  S2P_Joint_2/RConn1 -- Revolute_2_upper_arm_link/LConn2
  S2P_Joint_3/RConn1 -- Revolute_3_forearm_link/LConn2
  S2P_Joint_4/RConn1 -- Revolute_4_wrist_1_link/LConn2
  S2P_Joint_5/RConn1 -- Revolute_5_wrist_2_link/LConn2
  S2P_Joint_6/RConn1 -- Revolute_6_wrist_3_link/LConn2
